simulink model "sm_amrPioneer3DX_path_follow"  (R2025a)
settings: Solver=ode23t  StartTime=0.0  StopTime=35  RelTol=1e-3  AbsTol=1e-4
PostLoadFcn:
  | waypoints = [0 0; 4 2; 3 7; -3 6];
  | target_vel = 0.5;
  | lookahead_d = 2;
  | max_yaw_rate = 1;
StopFcn:
  | %robotPoses = out.yout{1}.Values.Data;
  | 
  | %figure(99);
  | %plot(waypoints(:,1), waypoints(:,2), 'k-x');
  | %hold all
  | %plot(robotPoses(:,1), robotPoses(:,2));
  | %title('XY Waypoint Tracking');
undefined symbols (not defined in the file or in its folder): X, Y, Z
libraries: sm_lib x100, nesl_utility x11, robotalgslib x1, simulink x1
(part 3 of 3)

== system sm_amrPioneer3DX_path_follow/Robot/WheelR/right_wheel ==
  Inertia : sm_lib/Body Elements/Inertia  InertiaType=Custom  Mass=0.1  MassUnits=kg  CenterOfMass=[0, 0, 0]  CenterOfMassUnits=m  MomentsOfInertia=[1, 1, 1]*0.01  MomentsOfInertiaUnits=kg*m^2  ProductsOfInertia=[0, 0, 0]  ProductsOfInertiaUnits=kg*m^2  GraphicType=None  MarkerShape=Inertia  MarkerSize=20  GraphicVisPropType=SimpleVisualProperties  GraphicDiffuseColor=[0.5 0.5 0.5]  GraphicOpacity=1.0  GraphicSpecularColor=[0.5 0.5 0.5 1.0]  GraphicAmbientColor=[0.15 0.15 0.15 1.0]  GraphicEmissiveColor=[0.0 0.0 0.0 1.0]  GraphicShininess=75
  InertiaOriginTransform : sm_lib/Frames and Transforms/Rigid Transform  RotationMethod=RotationSequence  FollAlignAxisA=+X  BaseAlignAxisA=+Y  FollAlignAxisB=+Y  BaseAlignAxisB=+Z  RotationStandardAxis=+Z  RotationAngle=0.0  RotationAngleUnits=deg  RotationArbitraryAxis=[0 0 1]  RotationSequenceAxes=BaseAxes  RotationSequence=XYZ  RotationSequenceAngles=[0, 0, 0]  RotationSequenceAnglesUnits=rad  RotationMatrix=[1 0 0; 0 1 0; 0 0 1]  Quaternion=[1 0 0 0]  TranslationMethod=Cartesian  TranslationCartesianOffset=[0, 0, 0]  TranslationCartesianOffsetUnits=m  TranslationStandardAxis=+Z  TranslationStandardOffset=0  TranslationStandardOffsetUnits=m  TranslationROffset=0  TranslationROffsetUnits=m  TranslationThetaOffset=0  TranslationThetaOffsetUnits=deg  TranslationZOffset=0  TranslationZOffsetUnits=m
  ReferenceFrame : sm_lib/Frames and Transforms/Reference Frame
  Spherical Solid For Contact : sm_lib/Body Elements/Spherical Solid  SphereRadius=0.0925  SphereRadiusUnits=m  ExportEntireGeometry=on  InertiaType=Custom  BasedOnType=Density  Density=1000  DensityUnits=kg/m^3  Mass=0  MassUnits=kg  CenterOfMass=[0 0 0]  CenterOfMassUnits=m  MomentsOfInertia=[0 0 0]  MomentsOfInertiaUnits=kg*m^2  ProductsOfInertia=[0 0 0]  ProductsOfInertiaUnits=kg*m^2  GraphicType=FromGeometry  MarkerShape=Sphere  MarkerSize=10  GraphicVisPropType=SimpleVisualProperties  GraphicDiffuseColor=clr_contact_sphere  GraphicOpacity=opc_contact_sphere  GraphicSpecularColor=[0.5 0.5 0.5 1.0]  GraphicAmbientColor=[0.15 0.15 0.15 1.0]  GraphicEmissiveColor=[0.0 0.0 0.0 1.0]  GraphicShininess=75  DoExposeReferenceFrame=on  SerializedFrames=<Frames/>
  Visual : sm_lib/Body Elements/File Solid  ExtGeomFileName=amr3dx_right_wheel.stl  UnitType=Custom  ExtGeomFileUnits=m  StepReaderType=HEX  ExportConvexHullGeometry=off  InertiaType=Custom  BasedOnType=DensityFromFile  Density=1000  DensityUnits=kg/m^3  Mass=0  MassUnits=kg  CenterOfMass=[0, 0, 0]  CenterOfMassUnits=m  MomentsOfInertia=[0, 0, 0]  MomentsOfInertiaUnits=kg*m^2  ProductsOfInertia=[0, 0, 0]  ProductsOfInertiaUnits=kg*m^2  GraphicType=FromGeometry  MarkerShape=Sphere  MarkerSize=10  GraphicVisPropType=SimpleVisualProperties  GraphicDiffuseColor=[0.117, 0.117, 0.117]  GraphicOpacity=1  GraphicSpecularColor=[0.5 0.5 0.5 1.0]  GraphicAmbientColor=[0.15 0.15 0.15 1.0]  GraphicEmissiveColor=[0.0 0.0 0.0 1.0]  GraphicShininess=75  DoExposeReferenceFrame=on  SerializedFrames=<Frames/>
  VisualOriginTransform : sm_lib/Frames and Transforms/Rigid Transform  RotationMethod=RotationSequence  FollAlignAxisA=+X  BaseAlignAxisA=+Y  FollAlignAxisB=+Y  BaseAlignAxisB=+Z  RotationStandardAxis=+Z  RotationAngle=0.0  RotationAngleUnits=deg  RotationArbitraryAxis=[0 0 1]  RotationSequenceAxes=BaseAxes  RotationSequence=XYZ  RotationSequenceAngles=[0, 0, 0]  RotationSequenceAnglesUnits=rad  RotationMatrix=[1 0 0; 0 1 0; 0 0 1]  Quaternion=[1 0 0 0]  TranslationMethod=Cartesian  TranslationCartesianOffset=[0, 0, 0]  TranslationCartesianOffsetUnits=m  TranslationStandardAxis=+Z  TranslationStandardOffset=0  TranslationStandardOffsetUnits=m  TranslationROffset=0  TranslationROffsetUnits=m  TranslationThetaOffset=0  TranslationThetaOffsetUnits=deg  TranslationZOffset=0  TranslationZOffsetUnits=m
  F : PMIOPort  Side=Left
  G : PMIOPort  Port=2  Side=Left
  connections:
  Inertia/RConn1 -- InertiaOriginTransform/RConn1
  ReferenceFrame/RConn1 -- F/RConn1 -- InertiaOriginTransform/LConn1 -- VisualOriginTransform/LConn1
  VisualOriginTransform/RConn1 -- Spherical Solid For Contact/RConn1 -- Visual/RConn1
  G/RConn1 -- Spherical Solid For Contact/LConn1

== matlab function sm_amrPioneer3DX_path_follow/Control/Wheel Speed Commands ==
  data: xy input; vCmd input; yawRateCmd input; waypoints input; wL output; stopThreshold input; slowThreshold input; trackWidth input; wheelRadius input; wR output
function [wL, wR] = wheelSpeed(xy, vCmd, yawRateCmd, waypoints, stopThreshold, slowThreshold,trackWidth,wheelRadius)

% Slow the robot down when it's near the threshold
distanceToEndpoint = norm(waypoints(end, :) - xy');
if (distanceToEndpoint < slowThreshold)
    vCmd = distanceToEndpoint/slowThreshold*vCmd;
    
    % Stop the robot if it's inside the target threshold
    if distanceToEndpoint < stopThreshold
        vCmd = 0;
    end
end

% Convert velocity and heading angular velocity to wheel speeds
wL = (vCmd - trackWidth/2*yawRateCmd)/wheelRadius;
wR = (vCmd + trackWidth/2*yawRateCmd)/wheelRadius;

end
